simulink model "Transmission_Line_Protection"  (R2024a)
settings: Solver=ode23tb  StartTime=0.0  StopTime=2.5  MaxStep=1e-5  RelTol=1e-4
libraries: spsRMSLib x6, spsThreePhaseBreakerLib x2, spsThreePhaseVIMeasurementLib x2, spsThreePhasePISectionLineLib x1, spsThreePhaseSeriesRLCLoadLib x1, spsThreePhaseFaultLib x1, spsThreePhaseSourceLib x1, sps_lib x1
settings Model: Creator=Admin  LastModifiedBy=Admin

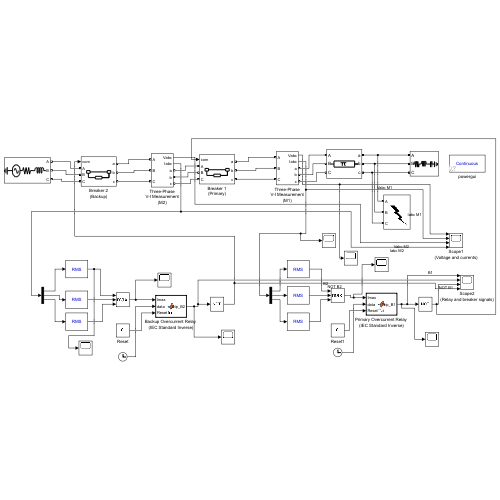
[thumbnail: Simulink's stored preview of the top-level diagram]
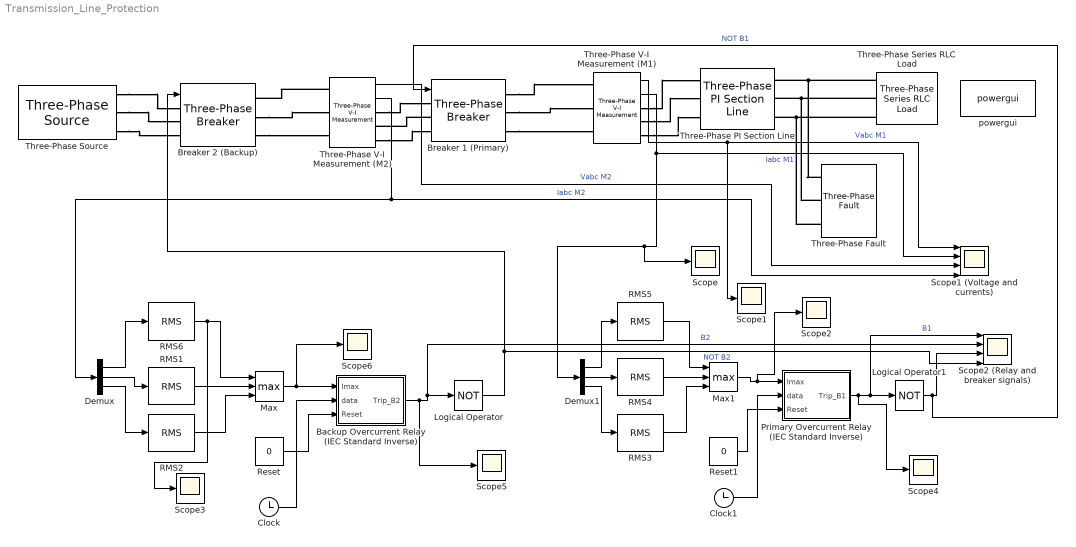
== system Transmission_Line_Protection ==
  Backup Overcurrent Relay (IEC Standard Inverse) : MATLAB Function  TreatAsAtomicUnit=on
  Breaker 1 (Primary) : spsThreePhaseBreakerLib/Three-Phase Breaker  InitialState=closed  SwitchA=on  SwitchB=on  SwitchC=on  SwitchTimes=[0.1 0.3]  External=on  BreakerResistance=0.01  SnubberResistance=1e6  SnubberCapacitance=inf  Measurements=None
  Breaker 2 (Backup) : spsThreePhaseBreakerLib/Three-Phase Breaker  InitialState=closed  SwitchA=on  SwitchB=on  SwitchC=on  SwitchTimes=[0.1 0.3]  External=on  BreakerResistance=0.01  SnubberResistance=1e6  SnubberCapacitance=inf  Measurements=None
  Clock : Clock
  Clock1 : Clock
  Demux : Demux  Outputs=3
  Demux1 : Demux  Outputs=3
  Logical Operator : Logic  Operator=NOT  AllPortsSameDT=off  OutDataTypeStr=boolean
  Logical Operator1 : Logic  Operator=NOT  AllPortsSameDT=off  OutDataTypeStr=boolean
  Max : MinMax  Function=max  Inputs=3
  Max1 : MinMax  Function=max  Inputs=3
  Primary Overcurrent Relay (IEC Standard Inverse) : MATLAB Function  TreatAsAtomicUnit=on
  RMS{1..6} (6 alike) : spsRMSLib/RMS  TrueRMS=on  Freq=50  RMSInit=120  Ts=0
  Reset : Constant  Value=0
  Reset1 : Constant  Value=0
  Scope{,1..6} (7 alike) : Scope
  Scope1 (Voltage and currents) : Scope  NumInputPorts=4
  Scope2 (Relay and breaker signals) : Scope  NumInputPorts=4
  Three-Phase PI Section Line : spsThreePhasePISectionLineLib/Three-Phase PI Section Line  LConnTagsString=a|b|c  RConnTagsString=A|B|C  Length=20  Frequency=50  Resistances=[ 0.01273 0.3864]  Inductances="[ 0.9337e-3  4.1264e-3]"  Capacitances=[12.74e-9 7.751e-9]
  Three-Phase Series RLC Load : spsThreePhaseSeriesRLCLoadLib/Three-Phase Series RLC Load  LConnTagsString=A|B|C  Configuration=Y (grounded)  NominalVoltage=11000  Vabc=[1e3 1e3 1e3]  Vabcp=[1e3 1e3 1e3]  NominalFrequency=50  UnbalancedPower=off  ActivePower=1.8e6  InductivePower=0.872e3  CapacitivePower=0.872e3  Pabc=[10e3 9e3 11e3]  QLabc=[100 90 110]  QCabc=[100 90 110]  Pabcp=[10e3 9e3 11e3]  QLabcp=[100 90 110]  QCabcp=[100 90 110]  Measurements=None  LoadType=constant Z
  Three-Phase V-I Measurement (M1) : spsThreePhaseVIMeasurementLib/Three-Phase V-I Measurement  VoltageMeasurement=phase-to-ground  SetLabelV=off  LabelV=Vabc  Vpu=off  VpuLL=off  CurrentMeasurement=yes  SetLabelI=off  LabelI=Iabc  Ipu=off  Pbase=100e6  Vbase=500e3  OutputType=Complex  PhasorSimulation=off  PSBequivalent=0
  Three-Phase V-I Measurement (M2) : spsThreePhaseVIMeasurementLib/Three-Phase V-I Measurement  VoltageMeasurement=phase-to-ground  SetLabelV=off  LabelV=Vabc  Vpu=off  VpuLL=off  CurrentMeasurement=yes  SetLabelI=off  LabelI=Iabc  Ipu=off  Pbase=100e6  Vbase=500e3  OutputType=Complex  PhasorSimulation=off  PSBequivalent=0
  Three-Phase Fault : spsThreePhaseFaultLib/Three-Phase Fault  InitialStates=0  FaultA=on  FaultB=on  FaultC=on  GroundFault=off  SwitchTimes=[0.1 2]  External=off  SwitchStatus=NaN  FaultResistance=0.01  GroundResistance=0.01  SnubberResistance=1e6  SnubberCapacitance=inf  Measurements=None
  Three-Phase Source : spsThreePhaseSourceLib/Three-Phase Source  InternalConnection=Yg  VoltagePhases=off  Voltage=11000  PhaseAngle=0  Voltage_phases=[25e3 25e3 25e3]/sqrt(3)  PhaseAngles_phases=[0 -120 +120]  Frequency=50  NonIdealSource=on  SpecifyImpedance=off  Resistance=0.1  Inductance=1e-3  ShortCircuitLevel=100e6  BaseVoltage=25e3  XRratio=7  BusType=swing  Pref=10e3  Qref=0  Prefabc=[10e3, 10e3, 10e3]  Qrefabc=[0, 0, 0]  Qmin=-inf  Qmax=inf
  powergui : sps_lib/powergui  Priority=1  SimulationMode=Continuous  SampleTime=50e-6  frequency=60  Iterations=50  frequencyindice=50  Pbase=100e6  ErrMax=1e-4  UnitsV=kV  UnitsW=MW  buscounter=0  FunctionMessages=off  echomessages=off  EnableUseOfTLC=off  CurrentSourceSwitches=off  DisableSnubberDevices=off  DisableRonSwitches=off  DisableVfSwitches=off  DisplayEquations=off  AutomaticDiscreteSolvers=off  SolverType=Tustin/Backward Euler (TBE)  Interpol=off  ExternalGateDelay=off  methode=off  Ts=100  x0status=blocks  SPID=on  SwTol=0  HookPort=off  NonlinearTolerance=1e-4  nMaxIteration=100  ContinueOnMaxIteration=off  RestoreLinks=warning  ResistiveCurrentMeasurement=off  Frange=[0:2:500]  Ylog=off  Xlog=on  ShowGrid=off  save=off  variable=ZData  structure=0  ZoomFFT=off  StartTime=0.0  cycles=1  DisplayStyle=1  fundamental=60  FreqAxis=off  MaxFrequency=1000  frequencyindicesteady=1  RmsSteady=1  display=off
  wires:
  Three-Phase V-I Measurement (M2)/2 -> Scope1 (Voltage and currents)/4, Demux/1  "Iabc M2"
  Demux/1 -> RMS6/1
  Demux/2 -> RMS1/1
  Demux/3 -> RMS2/1
  RMS6/1 -> Scope3/1, Max/1
  RMS1/1 -> Max/2
  RMS2/1 -> Max/3
  Three-Phase V-I Measurement (M1)/2 -> Scope/1, Demux1/1, Scope1 (Voltage and currents)/2  "Iabc M1"
  Demux1/1 -> RMS5/1
  Demux1/2 -> RMS4/1
  Demux1/3 -> RMS3/1
  RMS5/1 -> Max1/1
  RMS4/1 -> Max1/2
  RMS3/1 -> Max1/3
  Three-Phase V-I Measurement (M1)/1 -> Scope1/1, Scope1 (Voltage and currents)/1  "Vabc M1"
  Three-Phase V-I Measurement (M2)/1 -> Scope1 (Voltage and currents)/3  "Vabc M2"
  Reset/1 -> Backup Overcurrent Relay (IEC Standard Inverse)/3(Reset)
  Max1/1 -> Scope2/1, Primary Overcurrent Relay (IEC Standard Inverse)/1(Imax)
  Reset1/1 -> Primary Overcurrent Relay (IEC Standard Inverse)/3(Reset)
  Backup Overcurrent Relay (IEC Standard Inverse)/1(Trip_B2) -> Scope2 (Relay and breaker signals)/2, Logical Operator/1, Scope5/1  "B2"
  Primary Overcurrent Relay (IEC Standard Inverse)/1(Trip_B1) -> Scope4/1, Scope2 (Relay and breaker signals)/1, Logical Operator1/1  "B1"
  Logical Operator1/1 -> Scope2 (Relay and breaker signals)/3, Breaker 1 (Primary)/1  "NOT B1"
  Logical Operator/1 -> Scope2 (Relay and breaker signals)/4, Breaker 2 (Backup)/1  "NOT B2"
  Clock/1 -> Backup Overcurrent Relay (IEC Standard Inverse)/2(data)
  Clock1/1 -> Primary Overcurrent Relay (IEC Standard Inverse)/2(data)
  Max/1 -> Scope6/1, Backup Overcurrent Relay (IEC Standard Inverse)/1(Imax)
  connections:
  Three-Phase Source/RConn1 -- Breaker 2 (Backup)/LConn1
  Three-Phase Source/RConn2 -- Breaker 2 (Backup)/LConn2
  Three-Phase Source/RConn3 -- Breaker 2 (Backup)/LConn3
  Three-Phase V-I Measurement (M2)/LConn1 -- Breaker 2 (Backup)/RConn1
  Breaker 2 (Backup)/RConn2 -- Three-Phase V-I Measurement (M2)/LConn2
  Breaker 2 (Backup)/RConn3 -- Three-Phase V-I Measurement (M2)/LConn3
  Breaker 1 (Primary)/LConn2 -- Three-Phase V-I Measurement (M2)/RConn2
  Three-Phase V-I Measurement (M2)/RConn1 -- Breaker 1 (Primary)/LConn1
  Three-Phase V-I Measurement (M2)/RConn3 -- Breaker 1 (Primary)/LConn3
  Three-Phase Series RLC Load/LConn1 -- Three-Phase Fault/LConn1 -- Three-Phase PI Section Line/RConn1
  Three-Phase Series RLC Load/LConn2 -- Three-Phase Fault/LConn2 -- Three-Phase PI Section Line/RConn2
  Three-Phase Series RLC Load/LConn3 -- Three-Phase Fault/LConn3 -- Three-Phase PI Section Line/RConn3
  Breaker 1 (Primary)/RConn1 -- Three-Phase V-I Measurement (M1)/LConn1
  Breaker 1 (Primary)/RConn3 -- Three-Phase V-I Measurement (M1)/LConn3
  Breaker 1 (Primary)/RConn2 -- Three-Phase V-I Measurement (M1)/LConn2
  Three-Phase V-I Measurement (M1)/RConn1 -- Three-Phase PI Section Line/LConn1
  Three-Phase V-I Measurement (M1)/RConn2 -- Three-Phase PI Section Line/LConn2
  Three-Phase V-I Measurement (M1)/RConn3 -- Three-Phase PI Section Line/LConn3

== matlab function Transmission_Line_Protection/Primary Overcurrent Relay (IEC Standard Inverse) ==
  settings: updateMethod=DISCRETE
  data: Imax input; data input; Trip_B1 output; Reset input
function Trip_B1 = fcn(Imax, data, Reset)

persistent t trip
if isempty(t)
    t = 0;
    trip = 0;
end

Is = 125;
TMS = 0.10;
Ts = 1e-4;

if Reset ~= 0
    t = 0;
    trip = 0;
elseif Imax > Is && trip == 0
    t = t + Ts;
    M = Imax / Is;
    if t >= TMS*0.14/(M^0.02-1)
        trip = 1;
    end
else
    t = 0;
end

Trip_B1 = trip;

== matlab function Transmission_Line_Protection/Backup Overcurrent Relay (IEC Standard Inverse) ==
  settings: updateMethod=DISCRETE
  data: Imax input; data input; Trip_B2 output; Reset input
function Trip_B2 = fcn(Imax, data, Reset)

persistent startTime timing tripped

if isempty(tripped)
    startTime = 0;
    timing = false;
    tripped = false;
end

% Relay settings
Is = 125;       % Pickup current (A)
TMS = 0.25;     % Backup time multiplier

% Reset relay
if Reset ~= 0
    startTime = 0;
    timing = false;
    tripped = false;

elseif ~tripped

    if Imax > Is

        M = Imax / Is;

        % IEC Standard Inverse operating time
        tOp = 0.14*TMS/(M^0.02 - 1);

        if ~timing
            startTime = data;
            timing = true;
        end

        if (data - startTime) >= tOp
            tripped = true;
        end

    else
        startTime = 0;
        timing = false;
    end

end

Trip_B2 = double(tripped);

end
